simulink model "Controller_jtorque_cbf_22Franka"  (R2022b)
settings: Solver=FixedStepDiscrete  StartTime=0.0  StopTime=inf  FixedStep=0.001  RelTol=1e-3
PreLoadFcn:
  | set_param(gcs, 'RTWSystemTargetFile', 'franka_emika_panda.tlc');
  | 
  | demos_common_configs();
  | collision_behavior = ones(1,52)*100;
values from neighbouring files (symbols this model uses):
  b_sg = fliplr(B(end, :))    [init_joint_torque_cbf.m]
  cbf_dt = 0.001    [init_joint_torque_cbf.m]
  cbf_jtorque_params = [cbf_p_ths; cbf_v_ths; cbf_v_0; cbf_gamma; cbf_w_lin; cbf_w_slack;                        cbf_tau_limit; cbf_dt; plane_normal; plane_offset;                        cbf_latch_entry; cbf_zone_hyst; cbf_latch_alpha; cbf_tau_max;                        cbf_tau_rate; cbf_max_lat_force; cbf_max_moment;                        cbf_w_lateral; cbf_w_moment; cbf_w_null; cbf_guar_factor]    [init_joint_torque_cbf.m]
  cbf_Kd_rot = [120; 120; 120]*0    [init_joint_torque_cbf.m]
  cbf_Kd_trans = [2000; 2000; 0]*0    [init_joint_torque_cbf.m]
  cbf_stiff_decouple = 0    [init_joint_torque_cbf.m]
  cbf_zeta_rot = [0.7; 0.7; 0.7]*0    [init_joint_torque_cbf.m]
  cbf_zeta_trans = [0.7; 0.7; 0]*0    [init_joint_torque_cbf.m]
  Dn = 0 * ones(7,1)    [init_joint_torque_cbf.m]
  H_home = getTransform(Franka_robot, q_home, 'panda_link8', 'panda_link0')    [init_joint_torque_cbf.m]
  Kn = 0 * ones(7,1)    [init_joint_torque_cbf.m]
  plane_normal = [0.0; 0.0; 1.0]    [init_joint_torque_cbf.m]
  q_home = q_init    [init_joint_torque_cbf.m]
  q_init = [0 0  0  -(2/4)*pi  0  pi/2  -pi/4]'    [init_joint_torque_cbf.m]
undefined symbols (not defined in the file or in its folder): DiscIntNeverNeededParam, Fext_mag
libraries: franka_simulink_library x2, Robotics_lib x1, matrix_library x1
(part 1 of 7)
settings Model: SimulationMode=external  ExtModeTrigDuration=10000  Creator=vasi_ko  LastModifiedBy=rsladmin
settings SolverCC: AlgebraicLoopSolver=TrustRegion
settings DataIOCC: LimitDataPoints=on  SaveFormat=Array  ReturnWorkspaceOutputs=off
settings OptimizationCC: EnhancedBackFolding=on  OptimizeBlockOrder=speed  DifferentSizesBufferReuse=on  OptimizationCustomize=off
settings DebuggingCC: SolverPrmCheckMsg=warning  ParameterTunabilityLossMsg=error  UnconnectedInputMsg=warning  UnconnectedOutputMsg=warning  UnconnectedLineMsg=warning  SFUnexpectedBacktrackingDiag=warning  SFNoUnconditionalDefaultTransitionDiag=warning  SFExecutionAtInitializationDiag=none  SFMachineParentedDataDiag=warning  ArithmeticOperatorsInVariantConditions=warning
settings HardwareCC: ProdBitPerLong=64  ProdHWDeviceType=Intel->x86-64 (Linux 64)
settings ModelReferenceCC: EnableRefExpFcnMdlSchedulingChecks=on  PropagateSignalLabelsOutOfModel=off
settings SFSimCC: SimUseLocalCustomCode=off  MATLABDynamicMemAlloc=off  CustomCodeUndefinedFunction=UseInterfaceOnly  SimTargetLang=C++
settings RTWCC: SystemTargetFile=franka_emika_panda.tlc  RTWUseLocalCustomCode=off  CustomDefine=PINOCCHIO_WITH_URDFDOM  Toolchain=Franka Simulink | gmake (64-bit linux)  BuildConfiguration=Faster Runs  TargetLang=C++
settings RTWCC: CustomSource=|
  | /home/rsladmin/employees/parma/cbf_kinteach/joint_torque_cbf_controller/src/joint_torque_cbf_controller.cpp
  | /home/rsladmin/employees/parma/cbf_kinteach/cbf_common/src/profiles.cpp
settings RTWCC: CustomLibrary=|
  | /home/rsladmin/employees/parma/pinocchio_install/lib/libpinocchio.so
  | /usr/lib/x86_64-linux-gnu/libboost_filesystem.so
  | /usr/lib/x86_64-linux-gnu/libboost_serialization.so
  | /usr/lib/x86_64-linux-gnu/libboost_system.so
settings CodeAppCC: OperatorAnnotations=on
settings STFCustomTargetCC: TargetLangStandard=C99 (ISO)  ModelReferenceCompliant=off  MatFileLogging=on  GRTInterface=on  UseToolchainInfoCompliant=on  SystemTargetFile=franka_emika_panda.tlc
settings GRTTargetCC: ModelReferenceCompliant=off  ParMdlRefBuildCompliant=off  CompOptLevelCompliant=off  ConcurrentExecutionCompliant=off  CombineOutputUpdateFcns=off  CPPClassGenCompliant=off  GRTInterface=on  ExtModeStaticAlloc=on  ExtModeTransport=1  ExtModeMexFile=ext_xcp  ExtModeIntrfLevel=Level2 - Open
settings ConfigComp: CovMetricSettings=dw  CovSaveCumulativeToWorkspaceVar=on  CovSaveSingleToWorkspaceVar=on  CovExternalEMLEnable=off  CovSFcnEnable=off

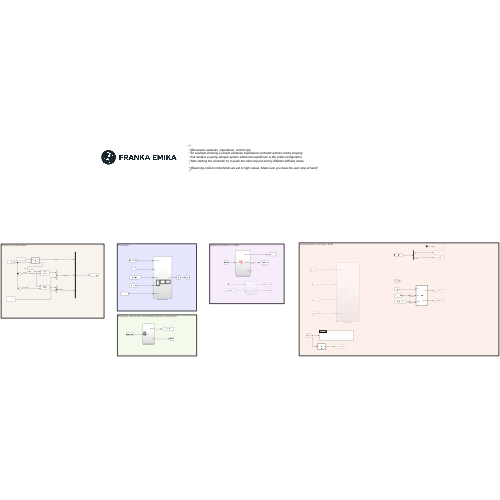
[thumbnail: Simulink's stored preview of the top-level diagram]
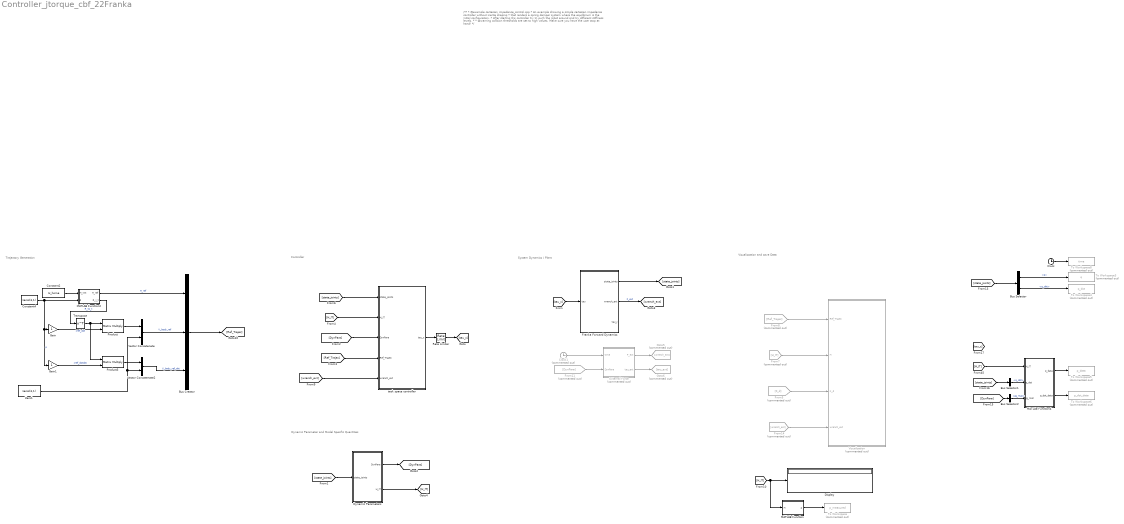
== system Controller_jtorque_cbf_22Franka ==
  note: /**
      |  * @example cartesian_impedance_control.cpp
      |  * An example showing a simple cartesian impedance controller without inertia shaping
      |  * that renders a spring damper system where the equilibrium is the initial configuration.
      |  * After starting the controller try to push the robot around and try different stiffness levels.
      |  *
      |  * @warning collision thresholds are set to high values. Make sure you have the user stop at hand!
      |  */
  note: Visualiszation and save Data
  note: Dynamic Parameter and Model Specific Quantities
  note: Controller
  note: System Dynamics / Plant
  note: Trajectory Generation
  Bus Creator : BusCreator  Inputs=3
  Bus Selector : BusSelector  OutputSignals=q,q_dot
  Bus Selector1 : BusSelector  OutputSignals=q_dot
  Bus Selector2 : BusSelector  OutputSignals=Jg_mat
  Clock : Clock
  Clock1 : Clock  Commented=on
  Constant2 : Constant  Value=H_home
  Constant4 : Constant  Value=zeros(3,1)
  Display : Display
  Dynamic Parameters : Subsystem
  External Force : Subsystem  Commented=on
  "Franka Forward Dynamics " : Subsystem
  From11 : From  Commented=on  GotoTag=DynPara
  From14 : From  Commented=on  GotoTag=wrench_ext
  From5 : From  Commented=on  GotoTag=K_d
  From7 : From  Commented=on  GotoTag=H_IT
  From8 : From  Commented=on  GotoTag=Ref_Trajec
  Gain : Gain
  Gain1 : Gain
  Goto5 : Goto  Commented=on  GotoTag=wrench_ext
  Goto6 : Goto  Commented=on  GotoTag=tau_ext
  MATLAB Function : MATLAB Function  TreatAsAtomicUnit=on
  MATLAB Function2 : MATLAB Function  TreatAsAtomicUnit=on
  MATLAB Function4 : MATLAB Function  TreatAsAtomicUnit=on
  Product : Product  Multiplication=Matrix(*)
  Product3 : Product  Multiplication=Matrix(*)
  Rate Limiter : RateLimiter  RisingSlewLimit=999  FallingSlewLimit=-999  SampleTimeMode=inherited
  To Workspace : ToWorkspace  Commented=on  VariableName=p_measured  SampleTime=-1
  To Workspace3 : ToWorkspace  Commented=on  VariableName=q  SampleTime=-1
  To Workspace4 : ToWorkspace  Commented=on  VariableName=q_dot  SampleTime=-1
  To Workspace5 : ToWorkspace  Commented=on  VariableName=p_data  SampleTime=-1
  To Workspace6 : ToWorkspace  Commented=on  VariableName=p_dot_data  SampleTime=-1
  To Workspace8 : ToWorkspace  Commented=on  VariableName=time  SampleTime=-1
  Transpose : Math  Operator=transpose
  Vector Concatenate : Concatenate
  Vector Concatenate2 : Concatenate
  Visualisation : Subsystem  Commented=on
  Zero1 : Constant  Value=zeros(3,1)  OutDataTypeStr=Inherit: Inherit via back propagation
  task space controller : Subsystem
  wires:
  From11/1 -> External Force/2(DynPara)
  [state_joints] -> task space controller/1(state_joints)
  Bus Selector/1 -> To Workspace3/1  "<q>"
  [DynPara] -> Bus Selector2/1
  Clock/1 -> To Workspace8/1
  External Force/2(tau_ext) -> Goto6/1
  From7/1 -> Visualisation/2(H)
  From14/1 -> Visualisation/4(wrench_ext)
  [DynPara] -> task space controller/3(DynPara)
  [H_IT] -> MATLAB Function4/1(H_IT)
  Clock1/1 -> External Force/1(time)
  External Force/1(F_ext) -> Goto5/1
  Bus Selector1/1 -> MATLAB Function4/2(q_dot)  "<q_dot>"
  [state_joints] -> Bus Selector1/1
  Dynamic Parameters/2(H_IT) -> [H_IT]
  From5/1 -> Visualisation/3(K_d)
  Rate Limiter/1 -> [tau_c]
  "Franka Forward Dynamics "/1(state_joints) -> [state_joints]
  task space controller/1(tau_c) -> Rate Limiter/1
  [state_joints] -> Bus Selector/1
  Dynamic Parameters/1(DynPara) -> [DynPara]
  MATLAB Function4/2(p_dot_data) -> To Workspace6/1
  [H_IT] -> task space controller/2(H_IT)
  Bus Selector2/1 -> MATLAB Function4/3(Jg_mat)  "<Jg_mat>"
  [wrench_ext] -> task space controller/5(wrench_ext)
  [Ref_Trajec] -> task space controller/4(Ref_Trajec)
  [H_IT] -> MATLAB Function/1(H), Display/1
  MATLAB Function4/1(p_data) -> To Workspace5/1
  From8/1 -> Visualisation/1(Ref_Trajec)
  MATLAB Function/1(p) -> To Workspace/1
  Bus Selector/2 -> To Workspace4/1  "<q_dot>"
  [state_joints] -> Dynamic Parameters/1(state_joints)
  [tau_c] -> "Franka Forward Dynamics "/1(tau)
  Bus Creator/1 -> [Ref_Trajec]
  Transpose/1 -> Product3/1, Product/1
  Zero1/1 -> Vector Concatenate/2, Vector Concatenate2/2
  Constant2/1 -> MATLAB Function2/1(H_init)
  Product/1 -> Vector Concatenate/1
  Gain1/1 -> Product3/2  "xref_dotdot"
  Vector Concatenate2/1 -> Bus Creator/3  "V_body_ref_dot"
  Constant4/1 -> Gain1/1, Gain/1, MATLAB Function2/2(d)  "p"
  Gain/1 -> Product/2  "xref_dot"
  Vector Concatenate/1 -> Bus Creator/2  "V_body_ref"
  MATLAB Function2/2(R_I_t) -> Transpose/1  "R_ts_t"
  MATLAB Function2/1(H_ref) -> Bus Creator/1  "H_ref"
  Product3/1 -> Vector Concatenate2/1
  "Franka Forward Dynamics "/2(wrench_ext) -> [wrench_ext]  "F_ext"

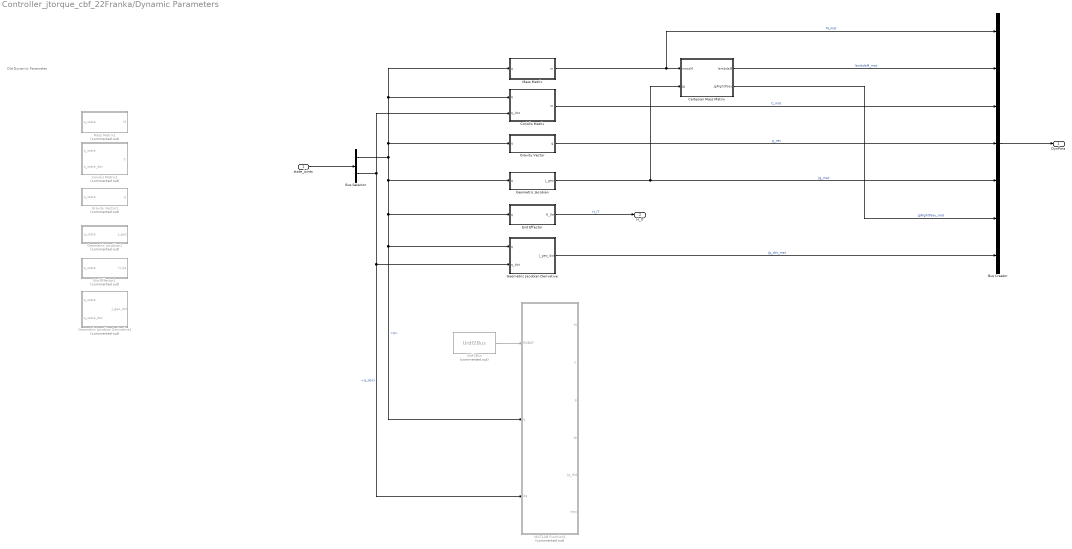
== system Controller_jtorque_cbf_22Franka/Dynamic Parameters ==
  note: Old Dynamic Parameter
  state_joints : Inport
  Bus Creator : BusCreator  Inputs=7
  Bus Selector : BusSelector  OutputSignals=q,q_dot
  Cartesian Mass Matrix : MATLAB Function  TreatAsAtomicUnit=on
  Coriolis Matrix : MATLAB Function  TreatAsAtomicUnit=on
  Coriolis Matrix1 : MATLAB Function  Commented=on  TreatAsAtomicUnit=on
  End Effector : MATLAB Function  TreatAsAtomicUnit=on
  End Effector1 : MATLAB Function  Commented=on  TreatAsAtomicUnit=on
  Geometric Jacobian : MATLAB Function  TreatAsAtomicUnit=on
  Geometric Jacobian Derivative : MATLAB Function  TreatAsAtomicUnit=on
  Geometric Jacobian Derivative1 : MATLAB Function  Commented=on  TreatAsAtomicUnit=on
  Geometric Jacobian1 : MATLAB Function  Commented=on  TreatAsAtomicUnit=on
  Gravity Vector : MATLAB Function  TreatAsAtomicUnit=on
  Gravity Vector1 : MATLAB Function  Commented=on  TreatAsAtomicUnit=on
  MATLAB Function1 : MATLAB Function  Commented=on  TreatAsAtomicUnit=on
  Mass Matrix : MATLAB Function  TreatAsAtomicUnit=on
  Mass Matrix1 : MATLAB Function  Commented=on  TreatAsAtomicUnit=on
  Urdf2Bus : Robotics_lib/Urdf2Bus  Commented=on  filename='Franka_arm.urdf'  tcp=9  S=[]
  DynPara : Outport
  H_IT : Outport  Port=2
  wires:
  state_joints/1 -> Bus Selector/1
  Urdf2Bus/1 -> MATLAB Function1/1(ROBOT)
  Bus Selector/1 -> Coriolis Matrix/1(q), Mass Matrix/1(q), Gravity Vector/1(q), Geometric Jacobian/1(q), MATLAB Function1/2(q), Geometric Jacobian Derivative/1(q), End Effector/1(q)  "<q>"
  Bus Selector/2 -> Geometric Jacobian Derivative/2(q_dot), MATLAB Function1/3(dq), Coriolis Matrix/2(q_dot)  "<q_dot>"
  Mass Matrix/1(m) -> Bus Creator/1, Cartesian Mass Matrix/1(massM)  "M_mat"
  Bus Creator/1 -> DynPara/1
  Cartesian Mass Matrix/1(lambdaM) -> Bus Creator/2  "lambdaM_mat"
  Coriolis Matrix/1(m) -> Bus Creator/3  "C_mat"
  Gravity Vector/1(g) -> Bus Creator/4  "g_vec"
  Cartesian Mass Matrix/2(JgRightPseu) -> Bus Creator/6  "JgRightPseu_mat"
  Geometric Jacobian Derivative/1(J_geo_dot) -> Bus Creator/7  "Jg_dot_mat"
  End Effector/1(H_0e) -> H_IT/1  "H_IT"
  Geometric Jacobian/1(J_geo) -> Cartesian Mass Matrix/2(Jg), Bus Creator/5  "Jg_mat"

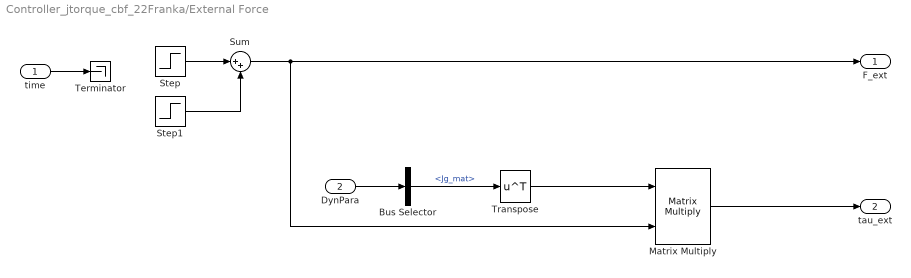
== system Controller_jtorque_cbf_22Franka/External Force ==
  time : Inport
  DynPara : Inport  Port=2
  Bus Selector : BusSelector  OutputSignals=Jg_mat
  Matrix Multiply : Product  Multiplication=Matrix(*)
  Step : Step  Time=5  Before=zeros(6,1)  After=Fext_mag.*[1;zeros(5,1)]  SampleTime=0
  Step1 : Step  Time=12  Before=zeros(6,1)  After=-Fext_mag.*[1;zeros(5,1)]  SampleTime=0
  Sum : Sum  Inputs=|++
  Terminator : Terminator
  Transpose : Math  Operator=transpose
  F_ext : Outport
  tau_ext : Outport  Port=2
  wires:
  Step/1 -> Sum/1
  Step1/1 -> Sum/2
  time/1 -> Terminator/1
  Sum/1 -> Matrix Multiply/2, F_ext/1
  Transpose/1 -> Matrix Multiply/1
  Bus Selector/1 -> Transpose/1  "<Jg_mat>"
  DynPara/1 -> Bus Selector/1
  Matrix Multiply/1 -> tau_ext/1

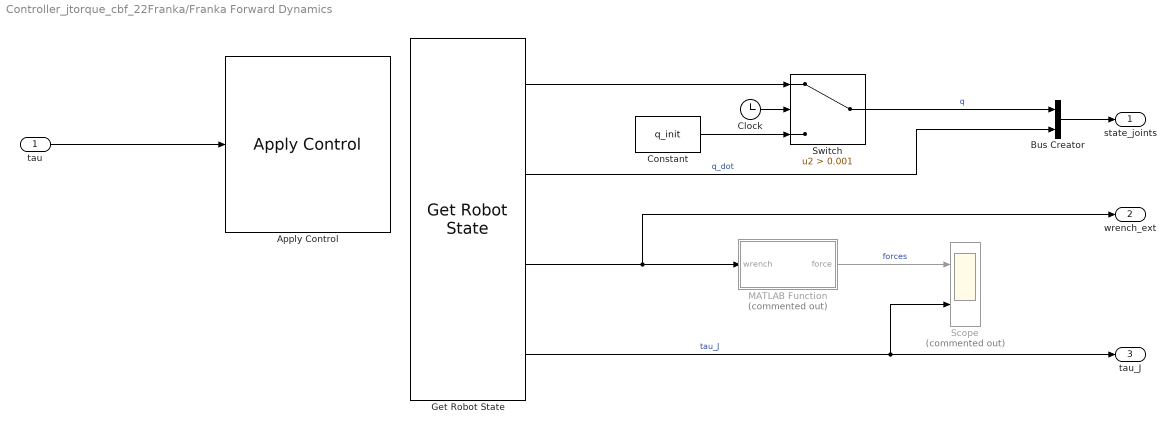
== system Controller_jtorque_cbf_22Franka/Franka Forward Dynamics  ==
  tau : Inport
  Apply Control : franka_simulink_library/Apply Control  robot_ip=robot_ip  gripper_attached=off  control_mode=Torque Control  controller_choice=Joint Impedance Controller  elbow_control=on  collision_thresholds=100*ones(1,52)  joint_impedance=joint_impedance  cartesian_impedance=cartesian_impedance  load_inertia=load_inertia  EE_T_K=EE_T_K  init_joint_configuration_req=on  init_joint_configuration=q_init'
      settings: SourceProductName=Franka Emika Simulink Support Package
  Bus Creator : BusCreator  Inputs=2
  Clock : Clock
  Constant : Constant  Value=q_init
  Get Robot State : franka_simulink_library/Get Robot State  robot_ip=robot_ip  signals_requested='q dq O_F_ext_hat_K tau_J'
      settings: SourceProductName=Franka Emika Simulink Support Package
  MATLAB Function : MATLAB Function  Commented=on  TreatAsAtomicUnit=on
  Scope : Scope  Commented=on  NumInputPorts=2
  Switch : Switch  Criteria=u2 > Threshold  Threshold=0.001  SaturateOnIntegerOverflow=off  InputSameDT=off
  state_joints : Outport
  wrench_ext : Outport  Port=2
  tau_J : Outport  Port=3
  wires:
  Get Robot State/2 -> Bus Creator/2  "q_dot"
  Get Robot State/1 -> Switch/1
  Get Robot State/3 -> wrench_ext/1, MATLAB Function/1(wrench)
  Constant/1 -> Switch/3
  Switch/1 -> Bus Creator/1  "q"
  Clock/1 -> Switch/2
  MATLAB Function/1(force) -> Scope/1  "forces"
  tau/1 -> Apply Control/1
  Bus Creator/1 -> state_joints/1
  Get Robot State/4 -> tau_J/1, Scope/2  "tau_J"

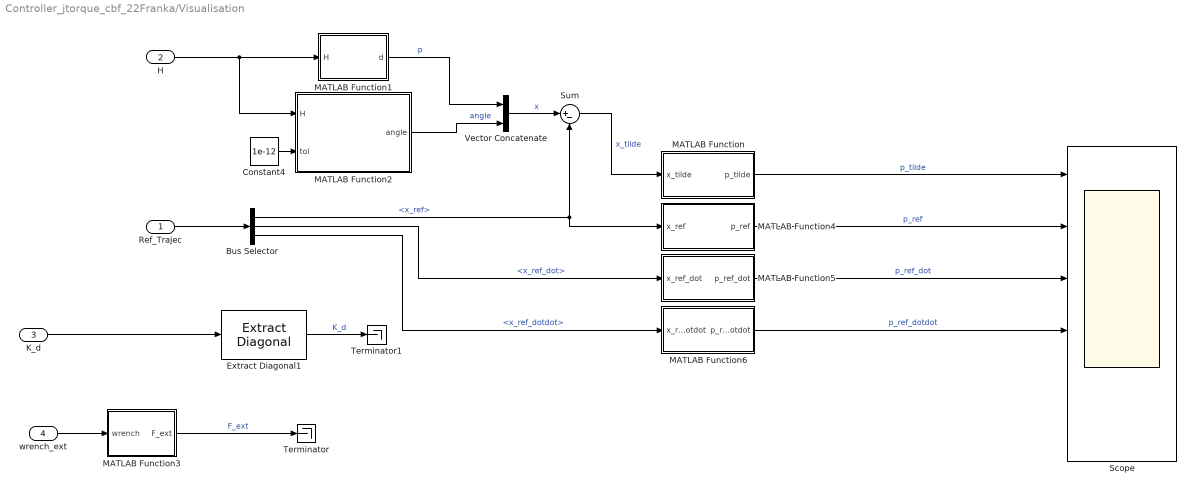
== system Controller_jtorque_cbf_22Franka/Visualisation ==
  Ref_Trajec : Inport
  H : Inport  Port=2
  K_d : Inport  Port=3
  wrench_ext : Inport  Port=4
  Bus Selector : BusSelector  OutputSignals=x_ref,x_ref_dot,x_ref_dotdot
  Constant4 : Constant  Value=1e-12
  Extract Diagonal1 : matrix_library/Extract Diagonal
      settings: LibrarySourceBlock=|
      | simulink/Matrix
      | Operations/Extract Diagonal
  MATLAB Function : MATLAB Function  TreatAsAtomicUnit=on
  MATLAB Function1 : MATLAB Function  TreatAsAtomicUnit=on
  MATLAB Function2 : MATLAB Function  TreatAsAtomicUnit=on
  MATLAB Function3 : MATLAB Function  TreatAsAtomicUnit=on
  MATLAB Function4 : MATLAB Function  TreatAsAtomicUnit=on
  MATLAB Function5 : MATLAB Function  TreatAsAtomicUnit=on
  MATLAB Function6 : MATLAB Function  TreatAsAtomicUnit=on
  Scope : Scope  NumInputPorts=6
  Sum : Sum  Inputs=|+-
  Terminator : Terminator
  Terminator1 : Terminator
  Vector Concatenate : Concatenate
  wires:
  H/1 -> MATLAB Function2/1(H), MATLAB Function1/1(H)
  MATLAB Function1/1(d) -> Vector Concatenate/1  "p"
  Ref_Trajec/1 -> Bus Selector/1
  Bus Selector/1 -> MATLAB Function4/1(x_ref), Sum/2  "<x_ref>"
  MATLAB Function/1(p_tilde) -> Scope/1  "p_tilde"
  Constant4/1 -> MATLAB Function2/2(tol)
  MATLAB Function2/1(angle) -> Vector Concatenate/2  "angle"
  Vector Concatenate/1 -> Sum/1  "x"
  Sum/1 -> MATLAB Function/1(x_tilde)  "x_tilde"
  Extract Diagonal1/1 -> Terminator1/1  "K_d"
  wrench_ext/1 -> MATLAB Function3/1(wrench)
  MATLAB Function3/1(F_ext) -> Terminator/1  "F_ext"
  K_d/1 -> Extract Diagonal1/1
  MATLAB Function4/1(p_ref) -> Scope/2  "p_ref"
  MATLAB Function5/1(p_ref_dot) -> Scope/3  "p_ref_dot"
  Bus Selector/2 -> MATLAB Function5/1(x_ref_dot)  "<x_ref_dot>"
  MATLAB Function6/1(p_ref_dotdot) -> Scope/4  "p_ref_dotdot"
  Bus Selector/3 -> MATLAB Function6/1(x_ref_dotdot)  "<x_ref_dotdot>"

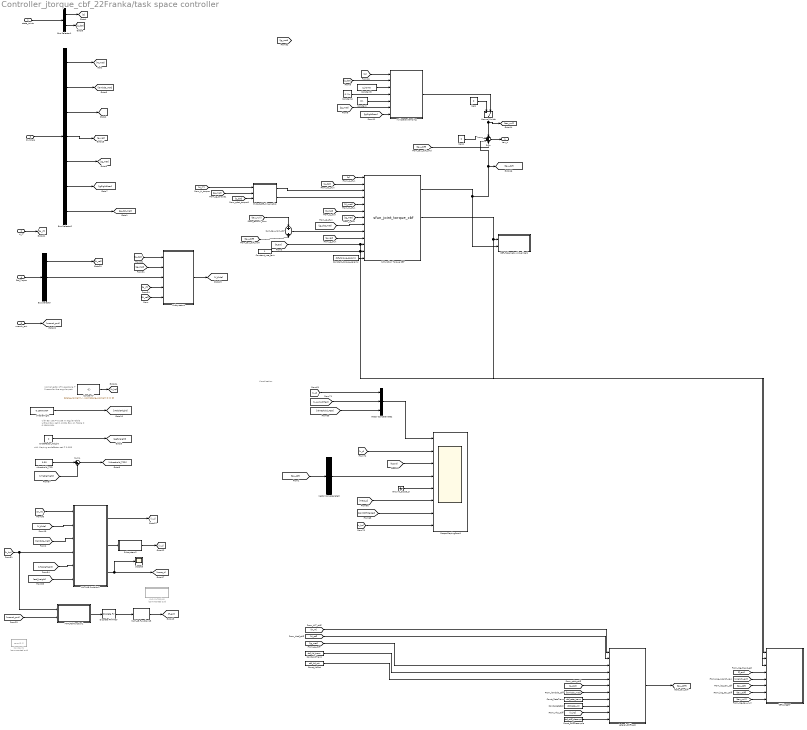
== system Controller_jtorque_cbf_22Franka/task space controller ==
  note: normalvector of hyperplane
      | + 3 zeros for the angular part
  note: with Box set = 0.106 m
      | regular table without box set = -0.004
      | Box on Table = 0.106-0.004
  note: with Waping endeffector set = 0.055
  note: Visualisation
  state_joints : Inport
  H_IT : Inport  Port=2
  DynPara : Inport  Port=3
  Ref_Trajec : Inport  Port=4
  wrench_ext : Inport  Port=5
  Bus Selector : BusSelector  OutputSignals=H_ref,V_body_ref,V_body_ref_dot
  Bus Selector1 : BusSelector  OutputSignals=q,q_dot
  Bus Selector2 : BusSelector  OutputSignals=M_mat,lambdaM_mat,C_mat,g_vec,Jg_mat,JgRightPseu_mat,Jg_dot_mat
  CBF_Logger : Subsystem
  CBF_Telemetry_Visualizer1 : Subsystem
      settings: PortSchema="{\"entries\":[{\"content\":{\"sides\":[{\"content\":{\"connectorIds\":[\"In1\",\"In2\"]},\"type\":\"ConnectorPlacement.EquallySpacedRectSide\",\"uuid\":\"710f47e5-147d-4a78-88ec-e281af76ee9f\"},{\"content\":{\"connectorIds\":[],\"side\":\"RIGHT\"},\"type\":\"ConnectorPlacement.EquallySpacedRectSide\",\"uuid\":\"9aa80510-4d6e-46c3-afa9-ad1226fbedc7\"},{\"content\":{\"connectorIds\":[],\"side\":\"TOP\"},\"type\":\"ConnectorPlacement.EquallySpacedRectSide\",\"uuid\":\"974fed3d-c6d1-41f4-ba7d-92d951d4e310\"},{\"content\":{\"connectorIds\":[\"In3\"],\"side\":\"BOTTOM\"},\"type\":\"ConnectorPlacement.EquallySpacedRectSide\",\"uuid\":\"a224dcdf-4876-4c61-a8a6-cdf7785f6603\"}]},\"type\":\"ConnectorPlacement.EquallySpacedConnector\",\"uuid\":\"a51230df-76b2-4a69-8099-ddb5762480b7\"}],\"packageUris\":[\"http://schema.mathworks.com/mf0/Connector/R2020b\"],\"version\":\"1.0\"}"
  Const_KdRot : Constant  Value=cbf_Kd_rot  VectorParams1D=off
  Const_KdTrans : Constant  Value=cbf_Kd_trans
  Const_StiffDecouple : Constant  Value=cbf_stiff_decouple
  Const_ZetaRot : Constant  Value=cbf_zeta_rot
  Const_ZetaTrans : Constant  Value=cbf_zeta_trans
  Constant : Constant  Value=Dn
  Constant1 : Constant  Commented=on  Value=zeros(3,1)
  Constant3 : Constant  Value=q_home
  Constant4 : Constant  Value=0.*Kn
  Constant7 : Constant  Value=[plane_normal(:)./norm(plane_normal); 0; 0; 0]  VectorParams1D=off
  Constant_torque_params : Constant  Value=cbf_jtorque_params
  Constant_use_fext : Constant
  Discrete FIR Filter : DiscreteFir  Coefficients=b_sg
  Extract_EE_Kinematics : MATLAB Function  TreatAsAtomicUnit=on
  Ground_Scope_5 : Ground
  Lateral_Stiffness : MATLAB Function  TreatAsAtomicUnit=on
  MATLAB Function1 : MATLAB Function  TreatAsAtomicUnit=on
  MATLAB Function15 : MATLAB Function  TreatAsAtomicUnit=on
  MATLAB Function2 : MATLAB Function  TreatAsAtomicUnit=on
  Manual Switch : ManualSwitch  CurrentSetting=0
  OLD FILTERiNG : Subsystem  Commented=on
  S-Function Torque CBF : S-Function  FunctionName=sfun_joint_torque_cbf  SFunctionDeploymentMode=off  EnableBusSupport=off
  Scope3 : Scope
  Scope:DapingPara1 : Scope  NumInputPorts=8
  Subsystem2 : Subsystem
  Subsystem4 : Subsystem
  Sum : Sum  Inputs=++++
  Sum4 : Sum  Inputs=|+-
  Sum_tau_nom_cbf : Sum
  Vector Concatenate2 : Concatenate  NumInputs=3
  Vector Concatenate3 : Concatenate  NumInputs=1
  Zero : Constant  Value=0  OutDataTypeStr=Inherit: Inherit via back propagation
  Zero1 : Constant  Value=0  OutDataTypeStr=Inherit: Inherit via back propagation
  endEffector_height : Constant  Value=0
  nullspace damping : MATLAB Function  TreatAsAtomicUnit=on
  xTableHight : Constant  Value=0.106-0.004
  xthreshold_TSD : Constant  Value=0.30
  tau_c : Outport
  wires:
  state_joints/1 -> Bus Selector1/1
  Sum/1 -> tau_c/1
  Constant/1 -> nullspace damping/5(Dn)
  Bus Selector/1 -> [H_ref]  "<H_ref>"
  Bus Selector/2 -> Subsystem4/3(V_body_ref)  "<V_body_ref>"
  nullspace damping/1(tau_nullspace) -> Manual Switch/2  "tau_null"
  Ref_Trajec/1 -> Bus Selector/1
  DynPara/1 -> Bus Selector2/1
  Bus Selector2/1 -> [M_mat]  "<M_mat>"
  Bus Selector2/3 -> [C_mat]  "<C_mat>"
  Bus Selector2/4 -> [g_vec]  "<g_vec>"
  [q] -> nullspace damping/1(q)
  Bus Selector2/5 -> [Jg_mat]  "<Jg_mat>"
  Bus Selector2/7 -> [Jg_dot_mat]  "<Jg_dot_mat>"
  [Jg_mat] -> nullspace damping/6(Jg)
  Bus Selector2/2 -> [lambda_mat]  "<lambdaM_mat>"
  Constant3/1 -> nullspace damping/3(q_ref)
  Constant4/1 -> nullspace damping/4(Kn)
  Bus Selector2/6 -> [JgRightPseu]  "<JgRightPseu_mat>"
  [JgRightPseu] -> nullspace damping/7(JgRightPseu)
  Bus Selector1/2 -> [q_dot]  "<q_dot>"
  [q_dot] -> nullspace damping/2(q_dot)
  Bus Selector1/1 -> [q]  "<q>"
  wrench_ext/1 -> [wrench_ext]
  Zero/1 -> Manual Switch/1
  xthreshold_TSD/1 -> Sum4/1
  [V_tilde] -> MATLAB Function2/2(V_tilde)
  [H_IT] -> MATLAB Function2/1(H_IT)
  [lambda_mat] -> MATLAB Function2/3(lambda_mat)
  xTableHight/1 -> [xTableHight]
  MATLAB Function2/1(x_c) -> [x_c]
  Subsystem2/1(x) -> [v_c]  "v_c"
  [q_dot] -> Subsystem4/1(q_dot)
  [Jg_mat] -> Subsystem4/2(Jg)
  Subsystem4/1(V_tilde) -> [V_tilde]
  [H_ref] -> Subsystem4/5(H_ref)
  H_IT/1 -> [H_IT]
  [H_IT] -> Subsystem4/4(Htm)
  Manual Switch/1 -> [tau_null], Sum/1
  endEffector_height/1 -> [eef_height]
  Constant7/1 -> [n_hp]
  MATLAB Function2/3(m_c) -> Scope3/1, [mass_c]
  [xTableHight] -> MATLAB Function2/5(xTableHight)
  [eef_height] -> MATLAB Function2/6(eef_height)
  [xTableHight] -> Sum4/2
  Sum4/1 -> [xthreshold_TSD]
  MATLAB Function2/2(v_c) -> Subsystem2/1(u)  "v_c"
  [x_c] -> Vector Concatenate2/1  "x_c"
  [xthreshold_TSD] -> Vector Concatenate2/3  "xthreshold_TSD"
  Vector Concatenate3/1 -> Scope:DapingPara1/4
  [pointOfIntersec] -> Scope:DapingPara1/7  "pointOfIntersec"
  [x_c_modified] -> Vector Concatenate2/2  "x_c_modified"
  [n_hp] -> Scope:DapingPara1/8  "n_hp"
  Vector Concatenate2/1 -> Scope:DapingPara1/1
  [mass_c] -> Scope:DapingPara1/6
  [v_c] -> Scope:DapingPara1/2  "v_c"
  [F_ext] -> Scope:DapingPara1/3
  Ground_Scope_5/1 -> Scope:DapingPara1/5
  Zero1/1 -> Sum/2
  MATLAB Function15/1(F) -> [F_ext]
  [n_hp] -> MATLAB Function1/1(n_hp), MATLAB Function2/4(n_hp)
  [wrench_ext] -> MATLAB Function1/2(wrench_ext)
  [tau_cbf] -> Vector Concatenate3/1
  Discrete FIR Filter/1 -> MATLAB Function15/1(u)
  MATLAB Function1/1(F_ext) -> Discrete FIR Filter/1
  [g_vec] -> S-Function Torque CBF/10
  S-Function Torque CBF/2 -> CBF_Telemetry_Visualizer1/1(telem), CBF_Logger/1(telemetry)
  [Jg_mat] -> Extract_EE_Kinematics/2(Jg)
  Constant_use_fext/1 -> S-Function Torque CBF/12, CBF_Logger/3(use_fext)
  [F_ext] -> S-Function Torque CBF/11, CBF_Logger/2(F_ext_cbf)
  [q] -> S-Function Torque CBF/1
  [H_IT] -> Extract_EE_Kinematics/1(H)
  [Jg_mat] -> S-Function Torque CBF/7
  S-Function Torque CBF/1 -> CBF_Telemetry_Visualizer1/2(tau_cbf), Sum/3, [tau_cbf]
  [M_mat] -> S-Function Torque CBF/5
  [C_mat] -> S-Function Torque CBF/6
  Extract_EE_Kinematics/2(v_ee) -> S-Function Torque CBF/4
  [q_dot] -> S-Function Torque CBF/2
  Extract_EE_Kinematics/1(x_ee) -> S-Function Torque CBF/3
  [Jg_dot_mat] -> S-Function Torque CBF/8
  Constant_torque_params/1 -> S-Function Torque CBF/13
  [q_dot] -> Extract_EE_Kinematics/3(q_dot)
  [F_ext] -> CBF_Logger/4(F_ext_est)
  [wrench_ext] -> CBF_Logger/5(wrench_raw)
  [tau_cbf] -> CBF_Logger/6(tau_cbf)
  [tau_stiff] -> CBF_Logger/7(tau_stiff)
  [tau_null] -> CBF_Logger/8(tau_null)
  [H_IT] -> Lateral_Stiffness/1(H_I_t)
  [H_ref] -> Lateral_Stiffness/2(H_I_D)
  [Jg_mat] -> Lateral_Stiffness/3(Jg)
  Const_KdTrans/1 -> Lateral_Stiffness/4(KdTrans)
  Const_KdRot/1 -> Lateral_Stiffness/5(KdRot)
  [q_dot] -> Lateral_Stiffness/6(q_dot)
  [lambda_mat] -> Lateral_Stiffness/7(Lambda)
  Const_ZetaTrans/1 -> Lateral_Stiffness/8(ZetaTrans)
  Const_ZetaRot/1 -> Lateral_Stiffness/9(ZetaRot)
  [n_hp] -> Lateral_Stiffness/10(n_hp)
  Const_StiffDecouple/1 -> Lateral_Stiffness/11(decouple)
  Lateral_Stiffness/1(tau_stiff) -> [tau_stiff]
  [tau_stiff] -> Sum/4
  Sum_tau_nom_cbf/1 -> S-Function Torque CBF/9
  [tau_null] -> Sum_tau_nom_cbf/1
  [tau_stiff] -> Sum_tau_nom_cbf/2

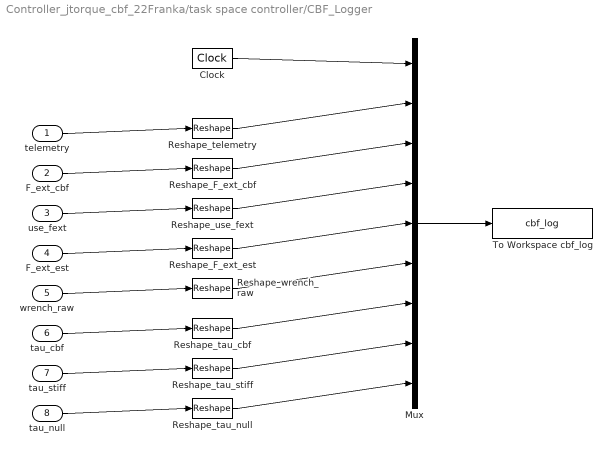
== system Controller_jtorque_cbf_22Franka/task space controller/CBF_Logger ==
  telemetry : Inport
  F_ext_cbf : Inport  Port=2
  use_fext : Inport  Port=3
  F_ext_est : Inport  Port=4
  wrench_raw : Inport  Port=5
  tau_cbf : Inport  Port=6
  tau_stiff : Inport  Port=7
  tau_null : Inport  Port=8
  Clock : DigitalClock  SampleTime=cbf_dt
  Mux : Mux  Inputs=9
  Reshape_F_ext_cbf : Reshape
  Reshape_F_ext_est : Reshape
  Reshape_tau_cbf : Reshape
  Reshape_tau_null : Reshape
  Reshape_tau_stiff : Reshape
  Reshape_telemetry : Reshape
  Reshape_use_fext : Reshape
  Reshape_wrench_raw : Reshape
  To Workspace cbf_log : ToWorkspace  VariableName=cbf_log  SampleTime=-1
      settings: Decimation=cbf_log_decimation
  wires:
  Clock/1 -> Mux/1
  telemetry/1 -> Reshape_telemetry/1
  Reshape_telemetry/1 -> Mux/2
  F_ext_cbf/1 -> Reshape_F_ext_cbf/1
  Reshape_F_ext_cbf/1 -> Mux/3
  use_fext/1 -> Reshape_use_fext/1
  Reshape_use_fext/1 -> Mux/4
  F_ext_est/1 -> Reshape_F_ext_est/1
  Reshape_F_ext_est/1 -> Mux/5
  wrench_raw/1 -> Reshape_wrench_raw/1
  Reshape_wrench_raw/1 -> Mux/6
  tau_cbf/1 -> Reshape_tau_cbf/1
  Reshape_tau_cbf/1 -> Mux/7
  tau_stiff/1 -> Reshape_tau_stiff/1
  Reshape_tau_stiff/1 -> Mux/8
  tau_null/1 -> Reshape_tau_null/1
  Reshape_tau_null/1 -> Mux/9
  Mux/1 -> To Workspace cbf_log/1

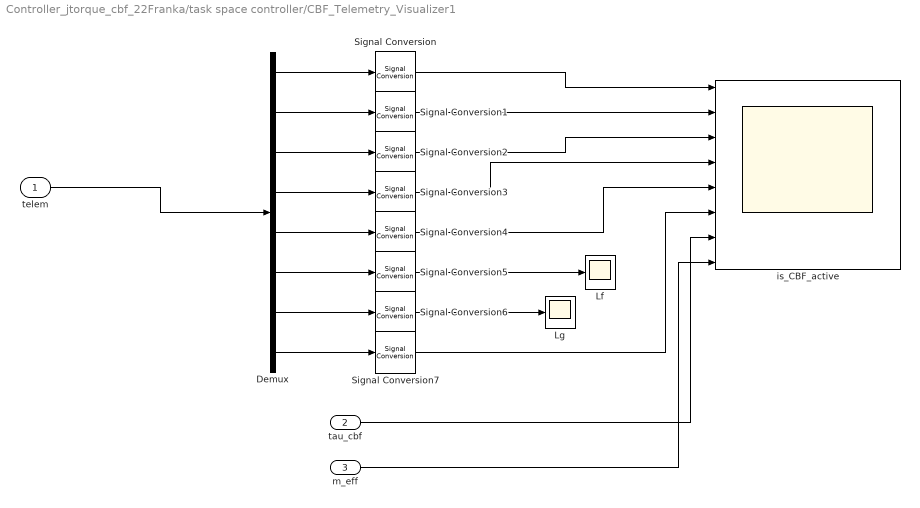
== system Controller_jtorque_cbf_22Franka/task space controller/CBF_Telemetry_Visualizer1 ==
  telem : Inport
  tau_cbf : Inport  Port=2
  m_eff : Inport  Port=3
  Demux : Demux  Outputs=8
  Lf : Scope
  Lg : Scope
  Signal Conversion{,1..7} (8 alike) : SignalConversion  OverrideOpt=off
  is_CBF_active : Scope  NumInputPorts=8
  wires:
  telem/1 -> Demux/1
  Demux/1 -> Signal Conversion/1
  Signal Conversion/1 -> is_CBF_active/1
  Signal Conversion1/1 -> is_CBF_active/2
  Demux/2 -> Signal Conversion1/1
  Signal Conversion2/1 -> is_CBF_active/3
  Demux/3 -> Signal Conversion2/1
  Signal Conversion3/1 -> is_CBF_active/4
  Demux/4 -> Signal Conversion3/1
  Signal Conversion4/1 -> is_CBF_active/5
  Demux/5 -> Signal Conversion4/1
  Signal Conversion5/1 -> Lf/1
  Demux/6 -> Signal Conversion5/1
  Signal Conversion6/1 -> Lg/1
  Demux/7 -> Signal Conversion6/1
  Signal Conversion7/1 -> is_CBF_active/6
  Demux/8 -> Signal Conversion7/1
  tau_cbf/1 -> is_CBF_active/7
  m_eff/1 -> is_CBF_active/8

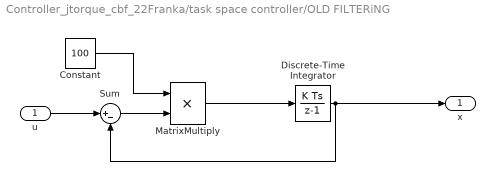
== system Controller_jtorque_cbf_22Franka/task space controller/OLD FILTERiNG ==
  u : Inport
  Constant : Constant  Value=100
  Discrete-Time Integrator : DiscreteIntegrator  SampleTime=-1  ICPrevOutput=DiscIntNeverNeededParam  ICPrevScaledInput=DiscIntNeverNeededParam
  MatrixMultiply : Product
  Sum : Sum  Inputs=|+-
  x : Outport
  wires:
  u/1 -> Sum/1
  Sum/1 -> MatrixMultiply/2
  Constant/1 -> MatrixMultiply/1
  MatrixMultiply/1 -> Discrete-Time Integrator/1
  Discrete-Time Integrator/1 -> Sum/2, x/1

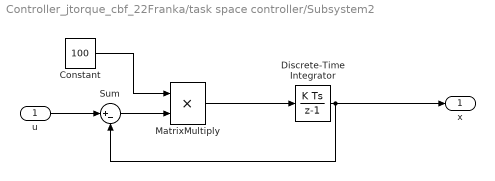
== system Controller_jtorque_cbf_22Franka/task space controller/Subsystem2 ==
  u : Inport
  Constant : Constant  Value=100
  Discrete-Time Integrator : DiscreteIntegrator  SampleTime=-1  ICPrevOutput=DiscIntNeverNeededParam  ICPrevScaledInput=DiscIntNeverNeededParam
  MatrixMultiply : Product
  Sum : Sum  Inputs=|+-
  x : Outport
  wires:
  u/1 -> Sum/1
  Sum/1 -> MatrixMultiply/2
  Constant/1 -> MatrixMultiply/1
  MatrixMultiply/1 -> Discrete-Time Integrator/1
  Discrete-Time Integrator/1 -> Sum/2, x/1

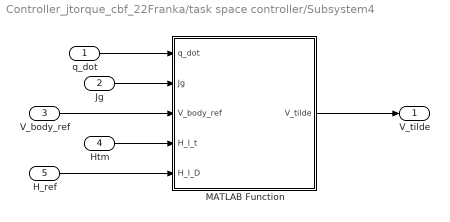
== system Controller_jtorque_cbf_22Franka/task space controller/Subsystem4 ==
  q_dot : Inport
  Jg : Inport  Port=2
  V_body_ref : Inport  Port=3
  Htm : Inport  Port=4
  H_ref : Inport  Port=5
  MATLAB Function : MATLAB Function  TreatAsAtomicUnit=on
  V_tilde : Outport
  wires:
  MATLAB Function/1(V_tilde) -> V_tilde/1
  Jg/1 -> MATLAB Function/2(Jg)
  q_dot/1 -> MATLAB Function/1(q_dot)
  Htm/1 -> MATLAB Function/4(H_I_t)
  H_ref/1 -> MATLAB Function/5(H_I_D)
  V_body_ref/1 -> MATLAB Function/3(V_body_ref)

== matlab function Controller_jtorque_cbf_22Franka/task space controller/MATLAB Function2 ==
  data: H_IT input; x_c output size=1; v_c output size=1; V_tilde input; lambda_mat input; n_hp input; m_c output size=1; xTableHight input; eef_height input
function [x_c, v_c, m_c] = fcn(H_IT, V_tilde, lambda_mat, n_hp, xTableHight, eef_height)

auxMat = zeros(4,4);
auxMat(3,4) = -xTableHight;

H = H_IT*[eye(3), [0;0;eef_height];zeros(1,3),1] + auxMat;

x_c = transpose(n_hp)*[H(1:3,4);zeros(3,1)];

v_c = transpose(n_hp)*V_tilde;




lambda_inv = lambda_mat\eye(6);
lambda_inv = (lambda_inv + transpose(lambda_inv))./2;

tmp3 = transpose(n_hp)*lambda_inv*n_hp;
m_c = tmp3\eye(1);


end

== matlab function Controller_jtorque_cbf_22Franka/Dynamic Parameters/End Effector ==
  data: q input; H_0e output
function H_0e = H_0e(q)
% Author: TU Wien, ACIN Robotics group
% Optimized and generated from Maple
  H_0e = zeros(4,4);
  t4449 = q(6);
  t4435 = sin(t4449);
  t4442 = cos(t4449);
  t4431 = 0.107e0 * t4435 + 0.88e-1 * t4442;
  t4450 = q(5);
  t4436 = sin(t4450);
  t4452 = q(3);
  t4438 = sin(t4452);
  t4491 = t4438 * t4436;
  t4499 = t4431 * t4491;
  t4430 = 0.107e0 * t4442 - 0.88e-1 * t4435 - 0.384e0;
  t4451 = q(4);
  t4437 = sin(t4451);
  t4498 = -t4430 * t4437 - 0.825e-1;
  t4443 = cos(t4450);
  t4427 = t4431 * t4443 - 0.825e-1;
  t4444 = cos(t4451);
  t4497 = t4427 * t4444;
  t4495 = t4430 * t4444;
  t4448 = q(7);
  t4434 = sin(t4448);
  t4454 = q(1);
  t4440 = sin(t4454);
  t4494 = t4434 * t4440;
  t4493 = t4436 * t4437;
  t4492 = t4437 * t4435;
  t4490 = t4438 * t4442;
  t4489 = t4438 * t4443;
  t4441 = cos(t4448);
  t4488 = t4440 * t4441;
  t4487 = t4443 * t4437;
  t4486 = t4443 * t4444;
  t4445 = cos(t4452);
  t4485 = t4443 * t4445;
  t4484 = t4444 * t4435;
  t4483 = t4445 * t4436;
  t4482 = t4445 * t4437;
  t4481 = t4445 * t4444;
  t4453 = q(2);
  t4439 = sin(t4453);
  t4446 = cos(t4453);
  t4467 = t4436 * t4481;
  t4458 = (t4467 + t4489) * t4446;
  t4478 = t4434 * t4493;
  t4480 = t4434 * t4458 + t4439 * t4478;
  t4479 = t4431 * t4483;
  t4477 = t4442 * t4487;
  t4476 = t4436 * t4490;
  t4475 = t4444 * t4491;
  t4474 = t4441 * t4493;
  t4473 = t4437 * t4490;
  t4472 = t4442 * t4486;
  t4471 = t4442 * t4483;
  t4470 = t4440 * t4485;
  t4469 = t4438 * t4486;
  t4468 = t4443 * t4481;
  t4466 = t4427 * t4437 + 0.316e0;
  t4465 = t4497 - t4498;
  t4464 = -0.1e1 * t4497 + t4498;
  t4463 = t4477 + t4484;
  t4462 = t4472 - 0.1e1 * t4492;
  t4461 = -0.1e1 * t4472 + t4492;
  t4460 = -0.1e1 * t4477 - 0.1e1 * t4484;
  t4459 = -0.1e1 * t4467 - 0.1e1 * t4489;
  t4447 = cos(t4454);
  t4457 = (t4475 - 0.1e1 * t4485) * t4447;
  t4456 = t4438 * t4462 + t4471;
  t4455 = -0.1e1 * t4471 + t4461 * t4438;
  t4425 = t4445 * t4461 + t4476;
  t4424 = t4462 * t4445 - 0.1e1 * t4476;
  t4423 = ((-0.1e1 * t4491 + t4468) * t4446 + t4439 * t4487) * t4435 + (t4446 * t4482 - 0.1e1 * t4439 * t4444) * t4442;
  t4422 = t4424 * t4446 + t4439 * t4463;
  t4421 = (t4425 * t4446 + t4439 * t4460) * t4434 + t4441 * t4458 + t4439 * t4474;
  t4420 = (t4465 * t4445 - 0.1e1 * t4499) * t4446 + (-0.1e1 * t4495 + t4466) * t4439;
  H_0e(1,3) = t4423 * t4447 + ((-0.1e1 * t4483 - 0.1e1 * t4469) * t4435 - 0.1e1 * t4473) * t4440;
  H_0e(4,1) = 0.0e0;
  H_0e(4,3) = 0.0e0;
  H_0e(3,1) = (t4425 * t4439 + t4446 * t4463) * t4441 + t4459 * t4434 * t4439 + t4446 * t4478;
  H_0e(2,1) = (t4422 * t4440 + t4447 * t4456) * t4441 + t4480 * t4440 + t4434 * t4457;
  H_0e(4,4) = 0.1e1;
  H_0e(3,2) = (t4424 * t4434 + t4441 * t4459) * t4439 + (t4434 * t4460 + t4474) * t4446;
  H_0e(3,4) = (t4445 * t4464 + t4499) * t4439 + 0.333e0 + (t4466 - t4495) * t4446;
  H_0e(2,3) = t4423 * t4440 + ((t4469 + t4483) * t4435 + t4473) * t4447;
  H_0e(2,4) = t4420 * t4440 + (t4438 * t4465 + t4479) * t4447;
  H_0e(4,2) = 0.0e0;
  H_0e(2,2) = t4434 * t4447 * t4455 + t4421 * t4440 + t4441 * t4457;
  H_0e(1,1) = (t4422 * t4441 + t4480) * t4447 + t4455 * t4488 - 0.1e1 * t4475 * t4494 + t4434 * t4470;
  H_0e(3,3) = ((t4491 - 0.1e1 * t4468) * t4435 - 0.1e1 * t4442 * t4482) * t4439 + (-0.1e1 * t4442 * t4444 + t4435 * t4487) * t4446;
  H_0e(1,4) = t4420 * t4447 + (-0.1e1 * t4479 + t4464 * t4438) * t4440;
  H_0e(1,2) = t4421 * t4447 + t4456 * t4494 - 0.1e1 * t4475 * t4488 + t4441 * t4470;
end

== matlab function Controller_jtorque_cbf_22Franka/Dynamic Parameters/End Effector1 ==
  data: q_state input; H_0e output
function H_0e = Franka_EndEffectorPos(q_state)
% Author: TU Wien, ACIN Robotics group
% Optimized and generated from Maple
  H_0e = zeros(4,4);

  t30 = q_state(6);
  t16 = sin(t30);
  t23 = cos(t30);
  t12 = 0.1070e0 * t16 + 0.88e-1 * t23;
  t31 = q_state(5);
  t17 = sin(t31);
  t33 = q_state(3);
  t19 = sin(t33);
  t71 = t19 * t17;
  t80 = t12 * t71;
  t11 = 0.1070e0 * t23 - 0.88e-1 * t16 - 0.384e0;
  t32 = q_state(4);
  t18 = sin(t32);
  t79 = -t11 * t18 - 0.825e-1;
  t25 = cos(t32);
  t24 = cos(t31);
  t8 = t12 * t24 - 0.825e-1;
  t78 = t8 * t25;
  t29 = q_state(7);
  t15 = sin(t29);
  t34 = q_state(2);
  t20 = sin(t34);
  t27 = cos(t34);
  t26 = cos(t33);
  t61 = t26 * t25;
  t57 = t17 * t61;
  t69 = t19 * t24;
  t39 = (t57 + t69) * t27;
  t72 = t17 * t18;
  t60 = t15 * t72;
  t77 = t15 * t39 + t20 * t60;
  t75 = t11 * t25;
  t35 = q_state(1);
  t21 = sin(t35);
  t74 = t15 * t21;
  t73 = t18 * t16;
  t70 = t19 * t23;
  t22 = cos(t29);
  t68 = t21 * t22;
  t67 = t24 * t18;
  t66 = t24 * t26;
  t65 = t16 * t25;
  t64 = t25 * t24;
  t63 = t26 * t17;
  t62 = t26 * t18;
  t59 = t12 * t63;
  t58 = t25 * t71;
  t56 = t17 * t70;
  t55 = t22 * t72;
  t54 = t18 * t70;
  t53 = t23 * t67;
  t52 = t23 * t64;
  t51 = t23 * t63;
  t50 = t21 * t66;
  t49 = t19 * t64;
  t48 = t24 * t61;
  t47 = t8 * t18 + 0.316e0;
  t46 = t78 - t79;
  t45 = t53 + t65;
  t44 = -0.1e1 * t73 + t52;
  t43 = -0.1e1 * t52 + t73;
  t42 = -0.1e1 * t78 + t79;
  t41 = -0.1e1 * t57 - 0.1e1 * t69;
  t40 = -0.1e1 * t53 - 0.1e1 * t65;
  t28 = cos(t35);
  t38 = (t58 - 0.1e1 * t66) * t28;
  t37 = t19 * t44 + t51;
  t36 = -0.1e1 * t51 + t43 * t19;
  t6 = t26 * t43 + t56;
  t5 = t44 * t26 - 0.1e1 * t56;
  t4 = ((-0.1e1 * t71 + t48) * t27 + t20 * t67) * t16 + (t27 * t62 - 0.1e1 * t20 * t25) * t23;
  t3 = t20 * t45 + t27 * t5;
  t2 = (t20 * t40 + t27 * t6) * t15 + t22 * t39 + t20 * t55;
  t1 = (t46 * t26 - 0.1e1 * t80) * t27 + (-0.1e1 * t75 + t47) * t20;
  H_0e(2,3) = t4 * t21 + ((t49 + t63) * t16 + t54) * t28;
  H_0e(3,3) = ((t71 - 0.1e1 * t48) * t16 - 0.1e1 * t23 * t62) * t20 + (t16 * t67 - 0.1e1 * t23 * t25) * t27;
%   H_0e(4,2) = 0.0e0;
  H_0e(2,4) = t1 * t21 + (t19 * t46 + t59) * t28;
%   H_0e(4,1) = 0.0e0;
  H_0e(2,2) = t15 * t28 * t36 + t2 * t21 + t22 * t38;
  H_0e(1,3) = t4 * t28 + ((-0.1e1 * t63 - 0.1e1 * t49) * t16 - 0.1e1 * t54) * t21;
  H_0e(1,2) = t2 * t28 + t37 * t74 - 0.1e1 * t58 * t68 + t22 * t50;
  H_0e(3,2) = (t15 * t5 + t22 * t41) * t20 + (t15 * t40 + t55) * t27;
  H_0e(1,4) = t1 * t28 + (-0.1e1 * t59 + t42 * t19) * t21;
  H_0e(1,1) = (t22 * t3 + t77) * t28 + t36 * t68 - 0.1e1 * t58 * t74 + t15 * t50;
  H_0e(2,1) = (t21 * t3 + t28 * t37) * t22 + t77 * t21 + t15 * t38;
  H_0e(4,4) = 1;
  H_0e(3,1) = (t20 * t6 + t27 * t45) * t22 + t41 * t15 * t20 + t27 * t60;
%   H_0e(4,3) = 0.0e0;
  H_0e(3,4) = (t26 * t42 + t80) * t20 + 0.333e0 + (t47 - t75) * t27;
end

== matlab function Controller_jtorque_cbf_22Franka/Dynamic Parameters/Geometric Jacobian ==
  data: q input; J_geo output
function J_geo = J_geometric(q)
% Author: TU Wien, ACIN Robotics group
% Optimized and generated from Maple
  J_geo = zeros(6,7);
  t4550 = q(3);
  t4544 = cos(t4550);
  t4549 = q(4);
  t4537 = sin(t4549);
  t4547 = q(6);
  t4535 = sin(t4547);
  t4532 = 0.88e-1 * t4535 + 0.384e0;
  t4541 = cos(t4547);
  t4571 = 0.107e0 * t4541;
  t4616 = -t4532 + t4571;
  t4621 = t4616 * t4537;
  t4513 = -0.825e-1 - t4621;
  t4543 = cos(t4549);
  t4584 = 0.88e-1 * t4541;
  t4527 = 0.107e0 * t4535 + t4584;
  t4548 = q(5);
  t4542 = cos(t4548);
  t4558 = t4527 * t4542 - 0.825e-1;
  t4610 = t4558 * t4543;
  t4623 = -t4610 + t4513;
  t4504 = t4623 * t4544;
  t4536 = sin(t4548);
  t4538 = sin(t4550);
  t4604 = t4538 * t4536;
  t4625 = t4527 * t4604 + t4504;
  t4567 = 0.10700e0 * t4535;
  t4514 = 0.82500e-1 + (-t4567 - t4584) * t4542;
  t4585 = 0.88e-1 * t4538;
  t4565 = t4536 * t4585;
  t4530 = t4541 * t4565;
  t4551 = q(2);
  t4539 = sin(t4551);
  t4545 = cos(t4551);
  t4560 = t4536 * t4567;
  t4615 = t4532 - 0.10700e0 * t4541;
  t4619 = ((t4514 * t4543 + t4537 * t4615 - 0.82500e-1) * t4544 + t4538 * t4560 + t4530) * t4539 + (-t4514 * t4537 + t4543 * t4615 + 0.316e0) * t4545;
  t4611 = t4558 * t4537;
  t4591 = t4545 * t4544;
  t4508 = (t4537 * t4539 + t4543 * t4591) * t4536 + t4545 * t4538 * t4542;
  t4552 = q(1);
  t4540 = sin(t4552);
  t4546 = cos(t4552);
  t4590 = t4546 * t4538;
  t4617 = t4536 * t4543 * t4590 + t4508 * t4540;
  t4606 = t4616 * t4543;
  t4554 = -t4606 + t4611;
  t4531 = 0.13375e2 * t4535 + 0.11e2 * t4541;
  t4613 = -0.8e-2 * t4531;
  t4570 = 0.107e0 * t4543;
  t4561 = t4542 * t4570;
  t4586 = 0.88e-1 * t4537;
  t4609 = (t4561 - t4586) * t4544;
  t4583 = 0.88e-1 * t4543;
  t4564 = t4542 * t4583;
  t4573 = 0.107e0 * t4537;
  t4608 = (t4564 + t4573) * t4544;
  t4605 = t4535 * t4537;
  t4603 = t4544 * t4539;
  t4602 = t4538 * t4540;
  t4601 = t4539 * t4540;
  t4600 = t4540 * t4543;
  t4599 = t4540 * t4544;
  t4598 = t4540 * t4545;
  t4597 = t4541 * t4537;
  t4596 = t4542 * t4539;
  t4595 = t4542 * t4543;
  t4594 = t4544 * t4536;
  t4593 = t4544 * t4543;
  t4592 = t4545 * t4537;
  t4589 = t4546 * t4539;
  t4588 = t4546 * t4544;
  t4519 = t4527 * t4594;
  t4582 = t4538 * t4600;
  t4581 = t4538 * t4596;
  t4580 = t4539 * t4593;
  t4579 = t4538 * t4597;
  t4578 = t4538 * t4595;
  t4577 = t4542 * t4593;
  t4576 = t4542 * t4588;
  t4575 = t4545 * t4590;
  t4574 = t4545 * t4588;
  t4572 = 0.107e0 * t4538;
  t4563 = 0.88e-1 * t4594;
  t4562 = t4536 * t4572;
  t4559 = -0.316e0 + t4606;
  t4556 = (-t4537 * t4585 + t4538 * t4561 + 0.107e0 * t4594) * t4541 - (t4537 * t4572 + t4538 * t4564 + t4563) * t4535;
  t4553 = (t4542 * t4573 + t4583) * t4541 + (-t4542 * t4586 + t4570) * t4535;
  t4533 = t4542 * t4599;
  t4503 = ((-0.1e1 * t4604 + t4577) * t4545 + t4537 * t4596) * t4535 + (t4537 * t4591 - 0.1e1 * t4539 * t4543) * t4541;
  t4502 = t4538 * t4623 - t4519;
  t4501 = -t4554 * t4591 + (t4610 + (t4571 - 0.1e1 * t4532) * t4537) * t4539;
  t4500 = ((-t4562 + t4609) * t4541 + (t4565 - 0.1e1 * t4608) * t4535) * t4545 + t4553 * t4539;
  J_geo(1,3) = t4502 * t4545 * t4546 + t4540 * t4625;
  J_geo(3,5) = 0.8e-2 * (t4581 + (t4580 - t4592) * t4536) * t4531;
  J_geo(6,4) = -0.1e1 * t4539 * t4538;
  J_geo(3,7) = 0.0e0;
  J_geo(4,1) = 0.0e0;
  J_geo(4,3) = t4589;
  J_geo(5,1) = 0.0e0;
  J_geo(5,6) = -0.1e1 * t4576 + t4617;
  J_geo(2,6) = t4500 * t4540 + t4546 * t4556;
  J_geo(4,5) = (-0.1e1 * t4574 + t4602) * t4537 + t4543 * t4589;
  J_geo(5,4) = t4538 * t4598 - 0.1e1 * t4588;
  J_geo(3,1) = 0.0e0;
  J_geo(6,3) = t4545;
  J_geo(4,7) = t4503 * t4546 + ((-0.1e1 * t4594 - 0.1e1 * t4578) * t4535 - 0.1e1 * t4579) * t4540;
  J_geo(6,7) = ((t4604 - 0.1e1 * t4577) * t4535 - 0.1e1 * t4544 * t4597) * t4539 + (-0.1e1 * t4543 * t4541 + t4542 * t4605) * t4545;
  J_geo(3,6) = ((t4562 - 0.1e1 * t4609) * t4541 + (-t4565 + t4608) * t4535) * t4539 + t4553 * t4545;
  J_geo(5,2) = t4546;
  J_geo(2,1) = (-t4625 * t4545 + (-0.1e1 * t4606 + t4611 + 0.316e0) * t4539) * t4546 - t4540 * t4519 - t4558 * t4582 + t4513 * t4602;
  J_geo(4,4) = t4575 + t4599;
  J_geo(5,5) = (-0.1e1 * t4540 * t4591 - 0.1e1 * t4590) * t4537 + t4539 * t4600;
  J_geo(6,5) = t4537 * t4603 + t4543 * t4545;
  J_geo(3,2) = (t4535 * t4562 + t4504 + t4530) * t4545 + (t4559 - t4611) * t4539;
  J_geo(3,4) = (t4621 + t4610) * t4545 + t4554 * t4603;
  J_geo(4,6) = t4508 * t4546 + t4533 - 0.1e1 * t4536 * t4582;
  J_geo(2,3) = t4502 * t4598 - t4546 * t4625;
  J_geo(2,7) = 0.0e0;
  J_geo(2,5) = (-t4576 + t4617) * t4613;
  J_geo(1,7) = 0.0e0;
  J_geo(2,4) = t4501 * t4540 - t4554 * t4590;
  J_geo(4,2) = -0.1e1 * t4540;
  J_geo(2,2) = t4540 * t4619;
  J_geo(1,1) = t4625 * t4598 + (-0.1e1 * t4519 + (-0.1e1 * t4610 + t4513) * t4538) * t4546 + (-0.1e1 * t4611 + t4559) * t4601;
  J_geo(5,3) = t4601;
  J_geo(6,1) = 0.1e1;
  J_geo(3,3) = (t4544 * t4560 - 0.1e1 * (-0.1e1 * t4541 * t4595 + t4605) * t4585 + t4563 * t4541 + (-0.384e0 * t4537 - 0.82500e-1 * t4543 + 0.82500e-1 + 0.10700e0 * t4535 * t4595 + 0.10700e0 * t4597) * t4538) * t4539;
  J_geo(5,7) = t4503 * t4540 + ((t4578 + t4594) * t4535 + t4579) * t4546;
  J_geo(1,5) = (t4542 * t4575 + t4533 + (t4537 * t4589 + (t4574 - t4602) * t4543) * t4536) * t4613;
  J_geo(6,2) = 0.0e0;
  J_geo(1,4) = t4501 * t4546 + t4554 * t4602;
  J_geo(1,2) = t4546 * t4619;
  J_geo(1,6) = t4500 * t4546 - t4540 * t4556;
  J_geo(6,6) = (-0.1e1 * t4580 + t4592) * t4536 - 0.1e1 * t4581;
end

== matlab function Controller_jtorque_cbf_22Franka/MATLAB Function4 ==
  data: H_IT input; p_data output; q_dot input; p_dot_data output; Jg_mat input
function [p_data, p_dot_data] = fcn(H_IT, q_dot, Jg_mat)

p_data = H_IT(1:3,4);

V = Jg_mat*q_dot;
p_dot_data = V(1:3);

end
